simulink model "fir_cosim_tb"  (R2026a)
settings: Solver=FixedStepDiscrete  StopTime=300  FixedStep=1
model workspace (MAT data in the model file):
  b = [0.125 0.375 0.375 0.125]
  f_noise = 0.4
  f_sig = 0.01
libraries: vivadosimlib x1
settings Model: Creator=KoayXianCong  LastModifiedBy=KoayXianCong

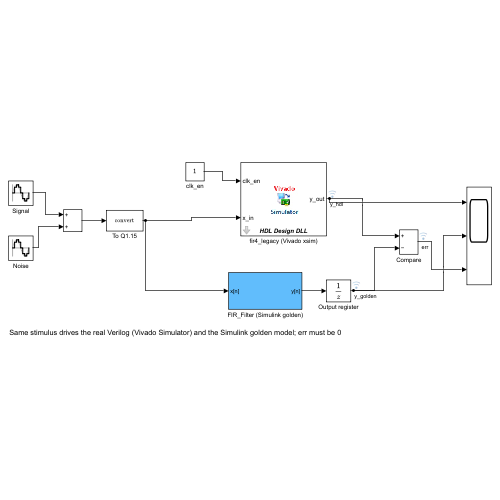
[thumbnail: Simulink's stored preview of the top-level diagram]
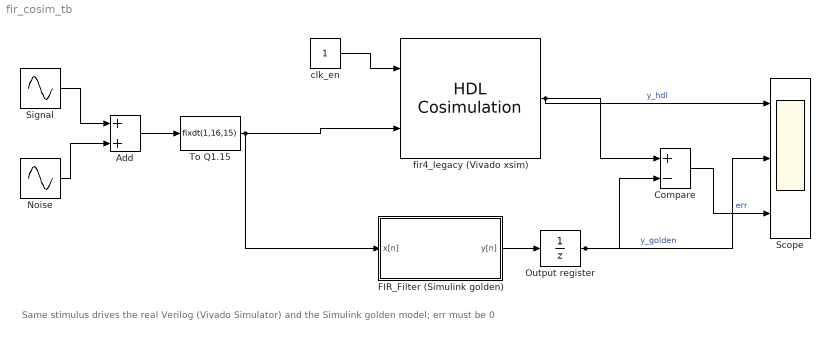
== system fir_cosim_tb ==
  note: Same stimulus drives the real Verilog (Vivado Simulator) and the Simulink golden model; err must be 0
  Add : Sum
  Compare : Sum  Inputs=+-
  FIR_Filter (Simulink golden) : Subsystem
  Noise : Sin  Amplitude=0.4  Frequency=2*pi*f_noise  SampleTime=1
  Output register : UnitDelay  SampleTime=-1
  Scope : Scope  NumInputPorts=3
      settings: TimeSpan=300
  Signal : Sin  Amplitude=0.5  Frequency=2*pi*f_sig  SampleTime=1
  To Q1.15 : DataTypeConversion  OutDataTypeStr=fixdt(1,16,15)  RndMeth=Nearest
  clk_en : Constant  OutDataTypeStr=boolean
  fir4_legacy (Vivado xsim) : vivadosimlib/HDL Cosimulation  PortPaths=/fir4_legacy/clk_en;/fir4_legacy/x_in;/fir4_legacy/y_out;  PortModes=[1 1 2 ]  PortTimes=[-1,-1,1]  PortSigns=[-1,-1,1,]  PortFracLengths=[0,0,18]  PortWordLengths=[-1,-1,19]  PortHDLWordSizes=[1,16,19]  CommLocal=on  CommSharedMemory=off  CommPortNumber=0  CommShowInfo=on  ClockPaths=/fir4_legacy/clk;/fir4_legacy/rst;  ClockModes=[2 3 ]  ClockTimes=[1e-08 8e-09 ]  TimingMode=ns  TimingScaleFactor=10  idxCellArray={'UNUSED_VAR'}  CosimBypass=Full Simulation  AllowDirectFeedthrough=on  ProductName=EDA Simulator Link VS  RunAutoTimescale=off  HdlClocks=/fir4_legacy/clk 10 ns;  PreRunTime=10  PreRunTimeUnit=ns
  wires:
  Signal/1 -> Add/1
  Noise/1 -> Add/2
  Add/1 -> To Q1.15/1
  clk_en/1 -> fir4_legacy (Vivado xsim)/1
  To Q1.15/1 -> fir4_legacy (Vivado xsim)/2, FIR_Filter (Simulink golden)/1(x[n])
  FIR_Filter (Simulink golden)/1(y[n]) -> Output register/1
  fir4_legacy (Vivado xsim)/1 -> Compare/1, Scope/1  "y_hdl"
  Output register/1 -> Compare/2, Scope/2  "y_golden"
  Compare/1 -> Scope/3  "err"

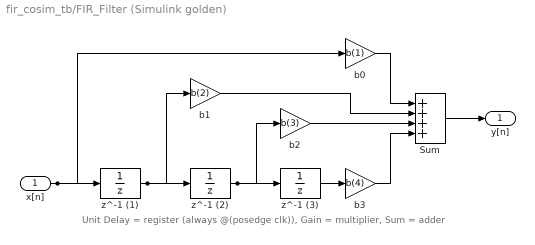
== system fir_cosim_tb/FIR_Filter (Simulink golden) ==
  note: Unit Delay = register (always @(posedge clk)), Gain = multiplier, Sum = adder
  x[n] : Inport
  Sum : Sum  Inputs=++++  OutDataTypeStr=fixdt(1,19,18)
  b0 : Gain  Gain=b(1)  ParamDataTypeStr=fixdt(1,16,15)
  b1 : Gain  Gain=b(2)  ParamDataTypeStr=fixdt(1,16,15)
  b2 : Gain  Gain=b(3)  ParamDataTypeStr=fixdt(1,16,15)
  b3 : Gain  Gain=b(4)  ParamDataTypeStr=fixdt(1,16,15)
  z^-1 (1) : UnitDelay  SampleTime=-1
  z^-1 (2) : UnitDelay  SampleTime=-1
  z^-1 (3) : UnitDelay  SampleTime=-1
  y[n] : Outport
  wires:
  Sum/1 -> y[n]/1
  b0/1 -> Sum/1
  z^-1 (3)/1 -> b3/1
  b3/1 -> Sum/4
  z^-1 (2)/1 -> b2/1, z^-1 (3)/1
  b2/1 -> Sum/3
  x[n]/1 -> z^-1 (1)/1, b0/1
  z^-1 (1)/1 -> b1/1, z^-1 (2)/1
  b1/1 -> Sum/2
